simulink model "snap_adc5g_spec"  (R2019a)
settings: Solver=VariableStepDiscrete  StartTime=0.0  StopTime=10.0  RelTol=1e-3
undefined symbols (not defined in the file): pfb_coeff_gen_calc
libraries: xbsIndex_r4 x13965, casper_library_misc x80, casper_library_delays x43, xps_library x5, xbsReplacements_r4 x2, casper_library_communications x1
(part 6 of 152)

== system snap_adc5g_spec/crosspower_vacc/detect_of1 ==
  in : Inport
  Constant2 : xbsIndex_r4/Constant  const=1  gui_display_data_type=Fixed-point  arith_type=Signed (2's comp)  n_bits=25  bin_pt=24  preci_type=Single  exp_width=8  frac_width=24  explicit_period=on  period=1  equ=P=C  opselect=C  inp2=PCIN>>17  opr=+  inp1=P  carry=CIN  dbl_ovrd=off  block_type=constant
  Constant4 : xbsIndex_r4/Constant  const=-1  gui_display_data_type=Fixed-point  arith_type=Signed (2's comp)  n_bits=25  bin_pt=24  preci_type=Single  exp_width=8  frac_width=24  explicit_period=on  period=1  equ=P=C  opselect=C  inp2=PCIN>>17  opr=+  inp1=P  carry=CIN  dbl_ovrd=off  block_type=constant
  Logical : xbsIndex_r4/Logical  logical_function=OR  inputs=2  en=off  latency=1  precision=Full  arith_type=Unsigned  n_bits=16  bin_pt=0  align_bp=on  dbl_ovrd=off  block_type=logical
  Relational2 : xbsIndex_r4/Relational  mode=a>=b  op_type=Bool  en=off  latency=1  dbl_ovrd=off  block_type=relational
  Relational4 : xbsIndex_r4/Relational  mode=a>=b  op_type=Bool  en=off  latency=1  dbl_ovrd=off  block_type=relational
  of : Outport
  wires:
  Relational4/1 -> Logical/2
  Constant4/1 -> Relational4/1
  Logical/1 -> of/1
  Relational2/1 -> Logical/1
  in/1 -> Relational4/2, Relational2/1
  Constant2/1 -> Relational2/2

== system snap_adc5g_spec/crosspower_vacc/detect_of2 ==
  in : Inport
  Constant2 : xbsIndex_r4/Constant  const=1  gui_display_data_type=Fixed-point  arith_type=Signed (2's comp)  n_bits=25  bin_pt=24  preci_type=Single  exp_width=8  frac_width=24  explicit_period=on  period=1  equ=P=C  opselect=C  inp2=PCIN>>17  opr=+  inp1=P  carry=CIN  dbl_ovrd=off  block_type=constant
  Constant4 : xbsIndex_r4/Constant  const=-1  gui_display_data_type=Fixed-point  arith_type=Signed (2's comp)  n_bits=25  bin_pt=24  preci_type=Single  exp_width=8  frac_width=24  explicit_period=on  period=1  equ=P=C  opselect=C  inp2=PCIN>>17  opr=+  inp1=P  carry=CIN  dbl_ovrd=off  block_type=constant
  Logical : xbsIndex_r4/Logical  logical_function=OR  inputs=2  en=off  latency=1  precision=Full  arith_type=Unsigned  n_bits=16  bin_pt=0  align_bp=on  dbl_ovrd=off  block_type=logical
  Relational2 : xbsIndex_r4/Relational  mode=a>=b  op_type=Bool  en=off  latency=1  dbl_ovrd=off  block_type=relational
  Relational4 : xbsIndex_r4/Relational  mode=a>=b  op_type=Bool  en=off  latency=1  dbl_ovrd=off  block_type=relational
  of : Outport
  wires:
  Relational4/1 -> Logical/2
  Constant4/1 -> Relational4/1
  Logical/1 -> of/1
  Relational2/1 -> Logical/1
  in/1 -> Relational4/2, Relational2/1
  Constant2/1 -> Relational2/2

== system snap_adc5g_spec/crosspower_vacc/detect_of3 ==
  in : Inport
  Constant2 : xbsIndex_r4/Constant  const=1  gui_display_data_type=Fixed-point  arith_type=Signed (2's comp)  n_bits=25  bin_pt=24  preci_type=Single  exp_width=8  frac_width=24  explicit_period=on  period=1  equ=P=C  opselect=C  inp2=PCIN>>17  opr=+  inp1=P  carry=CIN  dbl_ovrd=off  block_type=constant
  Constant4 : xbsIndex_r4/Constant  const=-1  gui_display_data_type=Fixed-point  arith_type=Signed (2's comp)  n_bits=25  bin_pt=24  preci_type=Single  exp_width=8  frac_width=24  explicit_period=on  period=1  equ=P=C  opselect=C  inp2=PCIN>>17  opr=+  inp1=P  carry=CIN  dbl_ovrd=off  block_type=constant
  Logical : xbsIndex_r4/Logical  logical_function=OR  inputs=2  en=off  latency=1  precision=Full  arith_type=Unsigned  n_bits=16  bin_pt=0  align_bp=on  dbl_ovrd=off  block_type=logical
  Relational2 : xbsIndex_r4/Relational  mode=a>=b  op_type=Bool  en=off  latency=1  dbl_ovrd=off  block_type=relational
  Relational4 : xbsIndex_r4/Relational  mode=a>=b  op_type=Bool  en=off  latency=1  dbl_ovrd=off  block_type=relational
  of : Outport
  wires:
  Relational4/1 -> Logical/2
  Constant4/1 -> Relational4/1
  Logical/1 -> of/1
  Relational2/1 -> Logical/1
  in/1 -> Relational4/2, Relational2/1
  Constant2/1 -> Relational2/2

== system snap_adc5g_spec/crosspower_vacc/of_count ==
  out_reg : Inport
  assert_reg : xbsIndex_r4/Assert  assert_type=on  type_source=Explicitly  gui_display_data_type=Fixed-point  arith_type=Unsigned  n_bits=32  bin_pt=0  preci_type=Single  exp_width=8  frac_width=24  assert_rate=off  rate_source=Explicitly  period=1  output_port=on  block_type=assert
  cast_gw : xbsIndex_r4/Convert  gui_display_data_type=Fixed-point  arith_type=Unsigned  n_bits=32  bin_pt=0  float_type=Single  exp_bits=8  fraction_bits=24  quantization=Truncate  overflow=Wrap  en=off  latency=1  pipeline=off  dbl_ovrd=off  block_type=convert
  io_delay : xbsIndex_r4/Delay  rst=off  infoeditControl=Selection of Reset will increase slice count due to use of real FFs and instead of SRLs  en=off  latency=0  reg_retiming=on  dbl_ovrd=off  block_type=delay
  reint1 : xbsIndex_r4/Reinterpret  force_arith_type=on  arith_type=Unsigned  force_bin_pt=on  bin_pt=0  block_type=reinterpret
  sim_out : Terminator
  sim_out_reg_gw : xbsIndex_r4/Gateway Out  inherit_from_input=off  hdl_port=off  rows=1  columns=1  UseAsDAC=off  DACChannel='1'  interface=None  automatic_assignment=on  address_offset=hex2dec('00')  intf_name=''  intf_description=''  timing_constraint=None  locs_specified=off  LOCs={}  io_standard={}  block_type=gatewayout
  sim_out_reg_sim_delay : xbsIndex_r4/Delay  rst=off  infoeditControl=Selection of Reset will increase slice count due to use of real FFs and instead of SRLs  en=off  latency=1  reg_retiming=on  dbl_ovrd=off  block_type=delay
  snap_adc5g_spec_crosspower_vacc_of_count_user_data_in : xbsIndex_r4/Gateway Out  inherit_from_input=off  hdl_port=on  rows=1  columns=1  UseAsDAC=off  DACChannel='1'  interface=None  automatic_assignment=on  address_offset=hex2dec('00')  intf_name=''  intf_description=''  timing_constraint=None  locs_specified=off  LOCs={}  io_standard={}  block_type=gatewayout
  sim_out_reg : Outport
  wires:
  sim_out_reg_sim_delay/1 -> sim_out_reg_gw/1
  sim_out_reg_gw/1 -> sim_out_reg/1
  io_delay/1 -> cast_gw/1
  cast_gw/1 -> snap_adc5g_spec_crosspower_vacc_of_count_user_data_in/1
  snap_adc5g_spec_crosspower_vacc_of_count_user_data_in/1 -> sim_out/1
  out_reg/1 -> sim_out_reg_sim_delay/1, assert_reg/1
  assert_reg/1 -> reint1/1
  reint1/1 -> io_delay/1

== system snap_adc5g_spec/crosspower_vacc/simple_bram_vacc ==
  new_acc : Inport
  din : Inport  Port=2
  Adder : xbsIndex_r4/AddSub  mode=Addition  use_carryin=off  use_carryout=off  en=off  latency=2  precision=User Defined  arith_type="Signed  (2's comp)"  n_bits=n_bits  bin_pt=bin_pt  quantization=Truncate  overflow=Wrap  use_behavioral_HDL=on  hw_selection=Fabric  pipelined=off  use_rpm=on  dbl_ovrd=off  block_type=addsub
      settings: xl_area=[0, 0, 0, 0, 0, 0, 0]  block_version=10.1.3
  Constant : xbsIndex_r4/Constant  const=0  gui_display_data_type=Fixed-point  arith_type=Signed (2's comp)  n_bits=n_bits  bin_pt=bin_pt  preci_type=Single  exp_width=8  frac_width=24  explicit_period=on  period=1  equ=P=C  opselect=C  inp2=PCIN>>17  opr=+  inp1=P  carry=CIN  dbl_ovrd=off  block_type=constant
  Mux : xbsIndex_r4/Mux  inputs=2  en=off  latency=0  precision=Full  arith_type="Signed  (2's comp)"  n_bits=8  bin_pt=2  quantization=Truncate  overflow=Wrap  dbl_ovrd=off  block_type=mux
      settings: xl_area=[0, 0, 0, 0, 0, 0, 0]
  delay_bram : Subsystem  mask(delay_bram){DelayLen=vec_len - 2, bram_latency=2}
      mask prompts: DelayLen "Delay By:"; bram_latency "BRAM Latency"
      mask help: A delay block that uses BRAM for its storage.
      mask init:
      | if (DelayLen <= bram_latency)
      | 	error('delay value must be greater than BRAM Latency');
      | end
      | BitWidth = max(ceil(log2(DelayLen)), 2);
      mask Help: eval('xlWeb(''http://casper.berkeley.edu/wiki/Delay_bram'')')
  pulse_ext : Subsystem  mask(pulse_ext){pulse_len=vec_len}
      mask prompts: pulse_len "Length of Pulse"
      mask help:
      | Extends a boolean signal to be high for the specified number of clocks after
      | the last high input.
      mask init:
      | bits = ceil(log2(pulse_len+1));
      mask Help: eval('xlWeb(''http://casper.berkeley.edu/wiki/Pulse_ext'')')
  dout : Outport
  valid : Outport  Port=2
  wires:
  Adder/1 -> delay_bram/1(In1)
  delay_bram/1(Out1) -> dout/1, Mux/2
  new_acc/1 -> pulse_ext/1(in)
  din/1 -> Adder/1
  pulse_ext/1(out) -> valid/1, Mux/1
  Mux/1 -> Adder/2
  Constant/1 -> Mux/3

== system snap_adc5g_spec/crosspower_vacc/simple_bram_vacc1 ==
  new_acc : Inport
  din : Inport  Port=2
  Adder : xbsIndex_r4/AddSub  mode=Addition  use_carryin=off  use_carryout=off  en=off  latency=2  precision=User Defined  arith_type="Signed  (2's comp)"  n_bits=n_bits  bin_pt=bin_pt  quantization=Truncate  overflow=Wrap  use_behavioral_HDL=on  hw_selection=Fabric  pipelined=off  use_rpm=on  dbl_ovrd=off  block_type=addsub
      settings: xl_area=[0, 0, 0, 0, 0, 0, 0]  block_version=10.1.3
  Constant : xbsIndex_r4/Constant  const=0  gui_display_data_type=Fixed-point  arith_type=Signed (2's comp)  n_bits=n_bits  bin_pt=bin_pt  preci_type=Single  exp_width=8  frac_width=24  explicit_period=on  period=1  equ=P=C  opselect=C  inp2=PCIN>>17  opr=+  inp1=P  carry=CIN  dbl_ovrd=off  block_type=constant
  Mux : xbsIndex_r4/Mux  inputs=2  en=off  latency=0  precision=Full  arith_type="Signed  (2's comp)"  n_bits=8  bin_pt=2  quantization=Truncate  overflow=Wrap  dbl_ovrd=off  block_type=mux
      settings: xl_area=[0, 0, 0, 0, 0, 0, 0]
  delay_bram : Subsystem  mask(delay_bram){DelayLen=vec_len - 2, bram_latency=2}
      mask prompts: DelayLen "Delay By:"; bram_latency "BRAM Latency"
      mask help: A delay block that uses BRAM for its storage.
      mask init:
      | if (DelayLen <= bram_latency)
      | 	error('delay value must be greater than BRAM Latency');
      | end
      | BitWidth = max(ceil(log2(DelayLen)), 2);
      mask Help: eval('xlWeb(''http://casper.berkeley.edu/wiki/Delay_bram'')')
  pulse_ext : Subsystem  mask(pulse_ext){pulse_len=vec_len}
      mask prompts: pulse_len "Length of Pulse"
      mask help:
      | Extends a boolean signal to be high for the specified number of clocks after
      | the last high input.
      mask init:
      | bits = ceil(log2(pulse_len+1));
      mask Help: eval('xlWeb(''http://casper.berkeley.edu/wiki/Pulse_ext'')')
  dout : Outport
  valid : Outport  Port=2
  wires:
  Adder/1 -> delay_bram/1(In1)
  delay_bram/1(Out1) -> dout/1, Mux/2
  new_acc/1 -> pulse_ext/1(in)
  din/1 -> Adder/1
  pulse_ext/1(out) -> valid/1, Mux/1
  Mux/1 -> Adder/2
  Constant/1 -> Mux/3

== system snap_adc5g_spec/crosspower_vacc/simple_bram_vacc2 ==
  new_acc : Inport
  din : Inport  Port=2
  Adder : xbsIndex_r4/AddSub  mode=Addition  use_carryin=off  use_carryout=off  en=off  latency=2  precision=User Defined  arith_type="Signed  (2's comp)"  n_bits=n_bits  bin_pt=bin_pt  quantization=Truncate  overflow=Wrap  use_behavioral_HDL=on  hw_selection=Fabric  pipelined=off  use_rpm=on  dbl_ovrd=off  block_type=addsub
      settings: xl_area=[0, 0, 0, 0, 0, 0, 0]  block_version=10.1.3
  Constant : xbsIndex_r4/Constant  const=0  gui_display_data_type=Fixed-point  arith_type=Signed (2's comp)  n_bits=n_bits  bin_pt=bin_pt  preci_type=Single  exp_width=8  frac_width=24  explicit_period=on  period=1  equ=P=C  opselect=C  inp2=PCIN>>17  opr=+  inp1=P  carry=CIN  dbl_ovrd=off  block_type=constant
  Mux : xbsIndex_r4/Mux  inputs=2  en=off  latency=0  precision=Full  arith_type="Signed  (2's comp)"  n_bits=8  bin_pt=2  quantization=Truncate  overflow=Wrap  dbl_ovrd=off  block_type=mux
      settings: xl_area=[0, 0, 0, 0, 0, 0, 0]
  delay_bram : Subsystem  mask(delay_bram){DelayLen=vec_len - 2, bram_latency=2}
      mask prompts: DelayLen "Delay By:"; bram_latency "BRAM Latency"
      mask help: A delay block that uses BRAM for its storage.
      mask init:
      | if (DelayLen <= bram_latency)
      | 	error('delay value must be greater than BRAM Latency');
      | end
      | BitWidth = max(ceil(log2(DelayLen)), 2);
      mask Help: eval('xlWeb(''http://casper.berkeley.edu/wiki/Delay_bram'')')
  pulse_ext : Subsystem  mask(pulse_ext){pulse_len=vec_len}
      mask prompts: pulse_len "Length of Pulse"
      mask help:
      | Extends a boolean signal to be high for the specified number of clocks after
      | the last high input.
      mask init:
      | bits = ceil(log2(pulse_len+1));
      mask Help: eval('xlWeb(''http://casper.berkeley.edu/wiki/Pulse_ext'')')
  dout : Outport
  valid : Outport  Port=2
  wires:
  Adder/1 -> delay_bram/1(In1)
  delay_bram/1(Out1) -> dout/1, Mux/2
  new_acc/1 -> pulse_ext/1(in)
  din/1 -> Adder/1
  pulse_ext/1(out) -> valid/1, Mux/1
  Mux/1 -> Adder/2
  Constant/1 -> Mux/3

== system snap_adc5g_spec/crosspower_vacc/simple_bram_vacc3 ==
  new_acc : Inport
  din : Inport  Port=2
  Adder : xbsIndex_r4/AddSub  mode=Addition  use_carryin=off  use_carryout=off  en=off  latency=2  precision=User Defined  arith_type="Signed  (2's comp)"  n_bits=n_bits  bin_pt=bin_pt  quantization=Truncate  overflow=Wrap  use_behavioral_HDL=on  hw_selection=Fabric  pipelined=off  use_rpm=on  dbl_ovrd=off  block_type=addsub
      settings: xl_area=[0, 0, 0, 0, 0, 0, 0]  block_version=10.1.3
  Constant : xbsIndex_r4/Constant  const=0  gui_display_data_type=Fixed-point  arith_type=Signed (2's comp)  n_bits=n_bits  bin_pt=bin_pt  preci_type=Single  exp_width=8  frac_width=24  explicit_period=on  period=1  equ=P=C  opselect=C  inp2=PCIN>>17  opr=+  inp1=P  carry=CIN  dbl_ovrd=off  block_type=constant
  Mux : xbsIndex_r4/Mux  inputs=2  en=off  latency=0  precision=Full  arith_type="Signed  (2's comp)"  n_bits=8  bin_pt=2  quantization=Truncate  overflow=Wrap  dbl_ovrd=off  block_type=mux
      settings: xl_area=[0, 0, 0, 0, 0, 0, 0]
  delay_bram : Subsystem  mask(delay_bram){DelayLen=vec_len - 2, bram_latency=2}
      mask prompts: DelayLen "Delay By:"; bram_latency "BRAM Latency"
      mask help: A delay block that uses BRAM for its storage.
      mask init:
      | if (DelayLen <= bram_latency)
      | 	error('delay value must be greater than BRAM Latency');
      | end
      | BitWidth = max(ceil(log2(DelayLen)), 2);
      mask Help: eval('xlWeb(''http://casper.berkeley.edu/wiki/Delay_bram'')')
  pulse_ext : Subsystem  mask(pulse_ext){pulse_len=vec_len}
      mask prompts: pulse_len "Length of Pulse"
      mask help:
      | Extends a boolean signal to be high for the specified number of clocks after
      | the last high input.
      mask init:
      | bits = ceil(log2(pulse_len+1));
      mask Help: eval('xlWeb(''http://casper.berkeley.edu/wiki/Pulse_ext'')')
  dout : Outport
  valid : Outport  Port=2
  wires:
  Adder/1 -> delay_bram/1(In1)
  delay_bram/1(Out1) -> dout/1, Mux/2
  new_acc/1 -> pulse_ext/1(in)
  din/1 -> Adder/1
  pulse_ext/1(out) -> valid/1, Mux/1
  Mux/1 -> Adder/2
  Constant/1 -> Mux/3

== system snap_adc5g_spec/fft_wideband_real/del_4x_pol0 ==
  d : Inport
  q : Outport
  wires:
  d/1 -> q/1

== system snap_adc5g_spec/fft_wideband_real/del_4x_pol1 ==
  d : Inport
  q : Outport
  wires:
  d/1 -> q/1

== system snap_adc5g_spec/fft_wideband_real/del_4x_pol2 ==
  d : Inport
  q : Outport
  wires:
  d/1 -> q/1

== system snap_adc5g_spec/fft_wideband_real/del_4x_pol3 ==
  d : Inport
  q : Outport
  wires:
  d/1 -> q/1

== system snap_adc5g_spec/fft_wideband_real/del_4x_pol4 ==
  d : Inport
  q : Outport
  wires:
  d/1 -> q/1

== system snap_adc5g_spec/fft_wideband_real/del_4x_pol5 ==
  d : Inport
  q : Outport
  wires:
  d/1 -> q/1

== system snap_adc5g_spec/fft_wideband_real/del_4x_pol6 ==
  d : Inport
  q : Outport
  wires:
  d/1 -> q/1

== system snap_adc5g_spec/fft_wideband_real/del_4x_pol7 ==
  d : Inport
  q : Outport
  wires:
  d/1 -> q/1

== system snap_adc5g_spec/fft_wideband_real/del_direct1 ==
  d : Inport
  q : Outport
  wires:
  d/1 -> q/1

== system snap_adc5g_spec/fft_wideband_real/del_direct2 ==
  d : Inport
  q : Outport
  wires:
  d/1 -> q/1

== system snap_adc5g_spec/fft_wideband_real/del_direct5 ==
  d : Inport
  q : Outport
  wires:
  d/1 -> q/1

== system snap_adc5g_spec/fft_wideband_real/del_direct6 ==
  d : Inport
  q : Outport
  wires:
  d/1 -> q/1

== system snap_adc5g_spec/fft_wideband_real/del_sync_4x ==
  d : Inport
  q : Outport
  wires:
  d/1 -> q/1

== system snap_adc5g_spec/fft_wideband_real/fft_biplex_real_4x ==
  sync : Inport
  shift : Inport  Port=2
  pol0_in : Inport  Port=3
  pol1_in : Inport  Port=4
  pol2_in : Inport  Port=5
  pol3_in : Inport  Port=6
  pol4_in : Inport  Port=7
  pol5_in : Inport  Port=8
  pol6_in : Inport  Port=9
  pol7_in : Inport  Port=10
  bi_real_unscr_4x : Subsystem  AncestorBlock=casper_library_ffts_internal/bi_real_unscr_4x  mask(bi_real_unscr_4x){n_inputs=2, FFTSize=11, n_bits=18, bin_pt=17, floating_point=off, float_type=single, exp_width=8, frac_width=24, add_latency=add_latency, conv_latency=conv_latency, bram_latency=bram_latency, bram_map=on, bram_delays=on, dsp48_adders=off, async=off}
      mask prompts: n_inputs "Number simultaneous inputs (2*?)"; FFTSize "Size of FFT (2^?):"; n_bits "Sample Bit Width"; bin_pt "Sample binary point"; floating_point "floating point"; float_type "float type"; exp_width "exponent width"; frac_width "fraction width"; add_latency "Add Latency"; conv_latency "Convert Latency"; bram_latency "BRAM Latency"; bram_map "Use BlockRAM for Map"; bram_delays "Use BlockRAM for Delays"; dsp48_adders "Use DSP48s for adders"; async "Asynchonrous operation"
      mask help: FFT internal block.
      mask init:
      | bi_real_unscr_4x_init(gcb, ...
      |     'n_inputs', n_inputs, ...
      |     'FFTSize', FFTSize, ...
      |     'n_bits', n_bits, ...
      |     'bin_pt', bin_pt, ...
      |     'floating_point', floating_point, ...
      |     'float_type', float_type, ...
      |     'exp_width', exp_width, ...
      |     'frac_width', frac_width, ...    
      |     'add_latency', add_latency, ...
      |     'conv_latency', conv_latency, ...
      |     'bram_latency', bram_latency, ...
      |     'bram_map', bram_map, ...
      |     'bram_delays', bram_delays, ...
      |     'dsp48_adders', dsp48_adders, ...
      |     'async', async);
      mask Callback floating_point:
      | onoff = get_param(gcb, 'floating_point');
      | if strcmp(onoff,'on')
      |     enable_fixpt = 'off'
      |     set_param_state(gcb, 'float_type', 'on')
      | 
      |     f_type = get_param(gcb, 'float_type')
      |     if strcmp(f_type,'custom')
      |         set_param_state(gcb, 'exp_width', 'on')
      |         set_param_state(gcb, 'frac_width', 'on')
      |     else
      |         set_param_state(gcb, 'exp_width', 'off')
      |         set_param_state(gcb, 'frac_width', 'off')
      |     end
      | 
      | 
      | else
      |     enable_fixpt = 'on'
      |     set_param_state(gcb, 'float_type', 'off')
      |     set_param_state(gcb, 'exp_width', 'off')
      |     set_param_state(gcb, 'frac_width', 'off')
      | end
      | 
      | set_param_state(gcb, 'n_bits', enable_fixpt)
      | set_param_state(gcb, 'bin_pt', enable_fixpt)
      mask TypeOptions float_type: single | custom
      mask Callback float_type:
      | f_type = get_param(gcb, 'float_type')
      | if strcmp(f_type,'custom')
      |     set_param_state(gcb, 'exp_width', 'on')
      |     set_param_state(gcb, 'frac_width', 'on')
      | else
      |     set_param_state(gcb, 'exp_width', 'off')
      |     set_param_state(gcb, 'frac_width', 'off')
      | end
      mask DialogControl ParameterTabVar0 Prompt: Basic
      mask DialogControl ParameterTabVar01 Prompt: Latency
      mask DialogControl ParameterTabVar012 Prompt: Implementation
  biplex_core : Subsystem  AncestorBlock=casper_library_ffts/biplex_core  mask(biplex_core){n_inputs=2, FFTSize=11, input_bit_width=18, bin_pt_in=17, coeff_bit_width=18, floating_point=off, float_type=single, exp_width=8, frac_width=24, add_latency=1, mult_latency=2, bram_latency=3, conv_latency=1, add_pipe_latency=0, mult_pipe_latency=0, quantization=Round  (unbiased: Even Values), overflow=Wrap, delays_bit_limit=8, coeffs_bit_limit=9, coeff_sharing=on, coeff_decimation=on, max_fanout=4, mult_spec=[2 2 2 2 2 2 2 2 2 2 2], bitgrowth=off, max_bits=19, hardcode_shifts=off, shift_schedule=[1 1 1 1 1 1 1 1 1 1 1], dsp48_adders=off, async=off}
      mask prompts: n_inputs "Number inputs (2*?)"; FFTSize "Size of FFT: (2^? pts)"; input_bit_width "Input Bit Width"; bin_pt_in "Input binary point"; coeff_bit_width "Coefficient Bit Width"; floating_point "floating point"; float_type "float type"; exp_width "exponent width"; frac_width "fraction width"; add_latency "Add Latency"; mult_latency "Mult Latency"; bram_latency "BRAM Latency"; conv_latency "Convert latency"; add_pipe_latency "Add Interface Pipeline Latency"; mult_pipe_latency "CMult Pipeline Latency"; quantization "Quantization Behavior"; overflow "Overflow Behavior"; delays_bit_limit "Number bits above which to implent stage's delays in BRAM (2^? bits)"; coeffs_bit_limit "Number bits above which to store stage's coefficients in BRAM (2^? bits)"; coeff_sharing "BRAM sharing in coeff storage"; coeff_decimation "Store a fraction of coeff factors where useful"; max_fanout "Maximum fanout"; mult_spec "Multiplier impl. (0=core, 1=embedded, 2=behavioural) (left=1st stage, or just one value)"; bitgrowth "Bit growth instead of shift"; max_bits "Maximum number of bits"; hardcode_shifts "Hardcode shift schedule"; shift_schedule "Shift schedule"; dsp48_adders "Use DSP48s for adders"; async "Asynchronous operation"
      mask help: FFT internal block.
      mask init:
      | biplex_core_init(gcb, ...
      |     'n_inputs', n_inputs, ...
      |     'FFTSize', FFTSize,...
      |     'input_bit_width', input_bit_width,...
      |     'bin_pt_in', bin_pt_in,...
      |     'coeff_bit_width', coeff_bit_width,...
      |     'floating_point', floating_point, ...
      |     'float_type', float_type, ...
      |     'exp_width', exp_width, ...
      |     'frac_width', frac_width, ...       
      |     'async', async, ...
      |     'add_latency', add_latency,...
      |     'mult_latency', mult_latency,...
      |     'bram_latency', bram_latency,...
      |     'conv_latency', conv_latency, ...
      |     'add_pipe_latency', add_pipe_latency, ...
      |     'mult_pipe_latency', mult_pipe_latency, ...        
      |     'quantization', quantization,...
      |     'overflow', overflow,...
      |     'delays_bit_limit', delays_bit_limit, ...
      |     'coeffs_bit_limit', coeffs_bit_limit, ...
      |     'coeff_sharing', coeff_sharing, ...
      |     'coeff_decimation', coeff_decimation, ...
      |     'max_fanout', max_fanout, ...
      |     'mult_spec', mult_spec, ...
      |     'bitgrowth', bitgrowth, ...
      |     'max_bits', max_bits, ...
      |     'hardcode_shifts', hardcode_shifts, ...
      |     'shift_schedule', shift_schedule, ...
      |     'dsp48_adders', dsp48_adders);
      settings: AttributesFormatString=11 stages
      mask Callback floating_point:
      | onoff = get_param(gcb, 'floating_point');
      | if strcmp(onoff,'on')
      |     enable_fixpt = 'off'
      |     set_param_state(gcb, 'float_type', 'on')
      | 
      |     f_type = get_param(gcb, 'float_type')
      |     if strcmp(f_type,'custom')
      |         set_param_state(gcb, 'exp_width', 'on')
      |         set_param_state(gcb, 'frac_width', 'on')
      |     else
      |         set_param_state(gcb, 'exp_width', 'off')
      |         set_param_state(gcb, 'frac_width', 'off')
      |     end
      | 
      | 
      | else
      |     enable_fixpt = 'on'
      |     set_param_state(gcb, 'float_type', 'off')
      |     set_param_state(gcb, 'exp_width', 'off')
      |     set_param_state(gcb, 'frac_width', 'off')
      | end
      | 
      | set_param_state(gcb, 'input_bit_width', enable_fixpt)
      | set_param_state(gcb, 'bin_pt_in', enable_fixpt)
      | set_param_state(gcb, 'coeff_bit_width', enable_fixpt)
      mask TypeOptions float_type: single | custom
      mask Callback float_type:
      | f_type = get_param(gcb, 'float_type')
      | if strcmp(f_type,'custom')
      |     set_param_state(gcb, 'exp_width', 'on')
      |     set_param_state(gcb, 'frac_width', 'on')
      | else
      |     set_param_state(gcb, 'exp_width', 'off')
      |     set_param_state(gcb, 'frac_width', 'off')
      | end
      mask TypeOptions quantization: Truncate | Round  (unbiased: +/- Inf) | Round  (unbiased: Even Values)
      mask TypeOptions overflow: Wrap | Saturate | Error
      mask Callback hardcode_shifts:
      | hardcode_shifts = get_param(gcb, 'hardcode_shifts');
      | set_param_state(gcb, 'shift_schedule', hardcode_shifts);
      mask Callback dsp48_adders: fft_callback_dsp48_adders(gcb);
      mask DialogControl ParameterTabVar0 Prompt: Basic
      mask DialogControl ParameterTabVar01 Prompt: Latency
      mask DialogControl ParameterTabVar012 Prompt: Implementation
  even_bussify : Subsystem  AncestorBlock=casper_library_flow_control/bus_create  mask(bus_create){inputNum=2}
      mask prompts: inputNum "Number of inputs:"
      mask init:
      | bus_create_init(gcb,...
      |     'inputNum', inputNum);
  odd_bussify : Subsystem  AncestorBlock=casper_library_flow_control/bus_create  mask(bus_create){inputNum=2}
      mask prompts: inputNum "Number of inputs:"
      mask init:
      | bus_create_init(gcb,...
      |     'inputNum', inputNum);
  pol0_debus : Subsystem  AncestorBlock=casper_library_flow_control/bus_expand  mask(bus_expand){mode=divisions of equal size, outputNum=2, outputWidth=36, outputBinaryPt=0, outputArithmeticType=0, show_format=off, outputToWorkspace=off, variablePrefix=out, outputToModelAsWell=on}
      mask prompts: outputNum "Number of outputs:"; outputWidth "Output width:"; outputBinaryPt "Output binary point position:"; outputArithmeticType "Output arithmetic type (ufix=0, fix=1, bool=2):"; show_format "Print format string?"; outputToWorkspace "Output to workspace?"; variablePrefix "Variable name prefix:"; outputToModelAsWell "Output to model as well?"
      mask help:
      | Expands a 'bus' made using a bus_create or Xilinx
      | concat block.
      | The input will be divided into the specified number
      | of outputs with the specified arithmetic types.
      | Divisions are made from most significant bit.
      mask init: same as snap_adc5g_spec/ss_adc/ctrl_split
      settings: AttributesFormatString=2 outputs
      mask TypeOptions mode: divisions of equal size | divisions of arbitrary size
      mask Callback mode: bus_expand_callback();
      mask Callback outputWidth: bus_expand_callback();
      mask Callback outputToWorkspace: bus_expand_callback();
  pol1_debus : Subsystem  AncestorBlock=casper_library_flow_control/bus_expand  mask(bus_expand){mode=divisions of equal size, outputNum=2, outputWidth=36, outputBinaryPt=0, outputArithmeticType=0, show_format=off, outputToWorkspace=off, variablePrefix=out, outputToModelAsWell=on}
      mask prompts: outputNum "Number of outputs:"; outputWidth "Output width:"; outputBinaryPt "Output binary point position:"; outputArithmeticType "Output arithmetic type (ufix=0, fix=1, bool=2):"; show_format "Print format string?"; outputToWorkspace "Output to workspace?"; variablePrefix "Variable name prefix:"; outputToModelAsWell "Output to model as well?"
      mask help:
      | Expands a 'bus' made using a bus_create or Xilinx
      | concat block.
      | The input will be divided into the specified number
      | of outputs with the specified arithmetic types.
      | Divisions are made from most significant bit.
      mask init: same as snap_adc5g_spec/ss_adc/ctrl_split
      settings: AttributesFormatString=2 outputs
      mask TypeOptions mode: divisions of equal size | divisions of arbitrary size
      mask Callback mode: bus_expand_callback();
      mask Callback outputWidth: bus_expand_callback();
      mask Callback outputToWorkspace: bus_expand_callback();
  pol2_debus : Subsystem  AncestorBlock=casper_library_flow_control/bus_expand  mask(bus_expand){mode=divisions of equal size, outputNum=2, outputWidth=36, outputBinaryPt=0, outputArithmeticType=0, show_format=off, outputToWorkspace=off, variablePrefix=out, outputToModelAsWell=on}
      mask prompts: outputNum "Number of outputs:"; outputWidth "Output width:"; outputBinaryPt "Output binary point position:"; outputArithmeticType "Output arithmetic type (ufix=0, fix=1, bool=2):"; show_format "Print format string?"; outputToWorkspace "Output to workspace?"; variablePrefix "Variable name prefix:"; outputToModelAsWell "Output to model as well?"
      mask help:
      | Expands a 'bus' made using a bus_create or Xilinx
      | concat block.
      | The input will be divided into the specified number
      | of outputs with the specified arithmetic types.
      | Divisions are made from most significant bit.
      mask init: same as snap_adc5g_spec/ss_adc/ctrl_split
      settings: AttributesFormatString=2 outputs
      mask TypeOptions mode: divisions of equal size | divisions of arbitrary size
      mask Callback mode: bus_expand_callback();
      mask Callback outputWidth: bus_expand_callback();
      mask Callback outputToWorkspace: bus_expand_callback();
  pol3_debus : Subsystem  AncestorBlock=casper_library_flow_control/bus_expand  mask(bus_expand){mode=divisions of equal size, outputNum=2, outputWidth=36, outputBinaryPt=0, outputArithmeticType=0, show_format=off, outputToWorkspace=off, variablePrefix=out, outputToModelAsWell=on}
      mask prompts: outputNum "Number of outputs:"; outputWidth "Output width:"; outputBinaryPt "Output binary point position:"; outputArithmeticType "Output arithmetic type (ufix=0, fix=1, bool=2):"; show_format "Print format string?"; outputToWorkspace "Output to workspace?"; variablePrefix "Variable name prefix:"; outputToModelAsWell "Output to model as well?"
      mask help:
      | Expands a 'bus' made using a bus_create or Xilinx
      | concat block.
      | The input will be divided into the specified number
      | of outputs with the specified arithmetic types.
      | Divisions are made from most significant bit.
      mask init: same as snap_adc5g_spec/ss_adc/ctrl_split
      settings: AttributesFormatString=2 outputs
      mask TypeOptions mode: divisions of equal size | divisions of arbitrary size
      mask Callback mode: bus_expand_callback();
      mask Callback outputWidth: bus_expand_callback();
      mask Callback outputToWorkspace: bus_expand_callback();
  ri_to_c0 : Subsystem  AncestorBlock=casper_library_misc/ri_to_c  mask(ri_to_c){}
      mask help:
      | Concatenates real and imaginary inputs into a complex output.
      | Useful for simplifying interconnects.
      | See also: Complex to Real-Imag (c_to_ri)
      mask Help: eval('xlWeb(''http://casper.berkeley.edu/wiki/Ri_to_c'')')
  ri_to_c1 : Subsystem  AncestorBlock=casper_library_misc/ri_to_c  mask(ri_to_c){}
      mask help:
      | Concatenates real and imaginary inputs into a complex output.
      | Useful for simplifying interconnects.
      | See also: Complex to Real-Imag (c_to_ri)
      mask Help: eval('xlWeb(''http://casper.berkeley.edu/wiki/Ri_to_c'')')
  ri_to_c2 : Subsystem  AncestorBlock=casper_library_misc/ri_to_c  mask(ri_to_c){}
      mask help:
      | Concatenates real and imaginary inputs into a complex output.
      | Useful for simplifying interconnects.
      | See also: Complex to Real-Imag (c_to_ri)
      mask Help: eval('xlWeb(''http://casper.berkeley.edu/wiki/Ri_to_c'')')
  ri_to_c3 : Subsystem  AncestorBlock=casper_library_misc/ri_to_c  mask(ri_to_c){}
      mask help:
      | Concatenates real and imaginary inputs into a complex output.
      | Useful for simplifying interconnects.
      | See also: Complex to Real-Imag (c_to_ri)
      mask Help: eval('xlWeb(''http://casper.berkeley.edu/wiki/Ri_to_c'')')
  sync_out : Outport
  pol0_out : Outport  Port=2
  pol1_out : Outport  Port=3
  pol2_out : Outport  Port=4
  pol3_out : Outport  Port=5
  pol4_out : Outport  Port=6
  pol5_out : Outport  Port=7
  pol6_out : Outport  Port=8
  pol7_out : Outport  Port=9
  of : Outport  Port=10
  wires:
  pol0_debus/1(msb_out2) -> pol0_out/1
  pol0_in/1 -> ri_to_c0/1(re)
  pol1_in/1 -> ri_to_c0/2(im)
  ri_to_c0/1(c) -> even_bussify/1(in1)
  pol1_debus/1(msb_out2) -> pol1_out/1
  pol2_debus/1(msb_out2) -> pol2_out/1
  pol2_in/1 -> ri_to_c1/1(re)
  pol3_in/1 -> ri_to_c1/2(im)
  ri_to_c1/1(c) -> odd_bussify/1(in1)
  pol3_debus/1(msb_out2) -> pol3_out/1
  pol0_debus/2(lsb_out1) -> pol4_out/1
  pol4_in/1 -> ri_to_c2/1(re)
  pol5_in/1 -> ri_to_c2/2(im)
  ri_to_c2/1(c) -> even_bussify/2(in2)
  pol1_debus/2(lsb_out1) -> pol5_out/1
  pol2_debus/2(lsb_out1) -> pol6_out/1
  pol6_in/1 -> ri_to_c3/1(re)
  pol7_in/1 -> ri_to_c3/2(im)
  ri_to_c3/1(c) -> odd_bussify/2(in2)
  pol3_debus/2(lsb_out1) -> pol7_out/1
  sync/1 -> biplex_core/1(sync)
  shift/1 -> biplex_core/2(shift)
  even_bussify/1(bus_out) -> biplex_core/3(pol1)
  odd_bussify/1(bus_out) -> biplex_core/4(pol2)
  biplex_core/4(of) -> of/1
  biplex_core/1(sync_out) -> bi_real_unscr_4x/1(sync)
  biplex_core/2(out1) -> bi_real_unscr_4x/2(even)
  biplex_core/3(out2) -> bi_real_unscr_4x/3(odd)
  bi_real_unscr_4x/1(sync_out) -> sync_out/1
  bi_real_unscr_4x/2(pol1_out) -> pol0_debus/1(bus_in)
  bi_real_unscr_4x/3(pol2_out) -> pol1_debus/1(bus_in)
  bi_real_unscr_4x/4(pol3_out) -> pol2_debus/1(bus_in)
  bi_real_unscr_4x/5(pol4_out) -> pol3_debus/1(bus_in)
